simulink model "SNS_GuiCircuit"  (R2025b)
settings: Solver=ode1  StartTime=0.0  StopTime=10.0  FixedStep=0.002  RelTol=1e-3
libraries: SNS_Library x9
Description:
  | SNS network generated from C:\Users\Ben\Documents\GitHub\Bipedal_Robot\Code\Matlab\SNS_Simscape\gui\circuit_last.json. u = input currents nA; S = MN drives in actuator order.
settings Model: Creator=Ben  LastModifiedBy=Ben

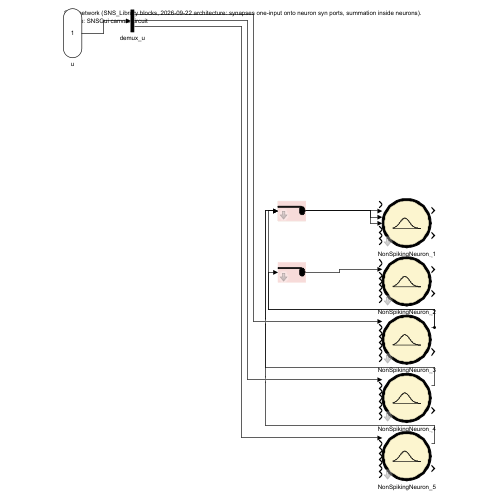
[thumbnail: Simulink's stored preview of the top-level diagram]
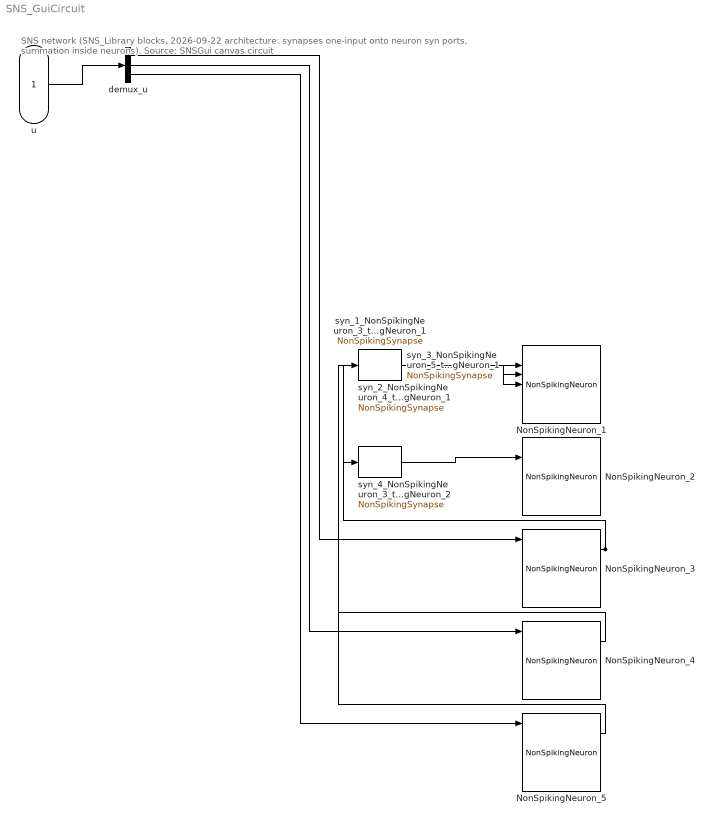
== system SNS_GuiCircuit ==
  note: SNS network (SNS_Library blocks, 2026-09-22 architecture: synapses one-input onto neuron syn ports, summation inside neurons).
      | Source: SNSGui canvas circuit
  u : Inport  PortDimensions=3
  NonSpikingNeuron_{1..5} (5 alike) : SNS_Library/NonSpikingNeuron  Vrest=-52  Gm=0.1  Cm=5  Thr=0  Slope=5
  demux_u : Demux  Outputs=3
  syn_1_NonSpikingNeuron_3_to_NonSpikingNeuron_1 : SNS_Library/NonSpikingSynapse  gmax=1  Esyn=0  ThrPre=-55  SlopePre=1
  syn_2_NonSpikingNeuron_4_to_NonSpikingNeuron_1 : SNS_Library/NonSpikingSynapse  gmax=1  Esyn=-72  ThrPre=-55  SlopePre=1
  syn_3_NonSpikingNeuron_5_to_NonSpikingNeuron_1 : SNS_Library/NonSpikingSynapse  gmax=1  Esyn=-72  ThrPre=-55  SlopePre=1
  syn_4_NonSpikingNeuron_3_to_NonSpikingNeuron_2 : SNS_Library/NonSpikingSynapse  gmax=1  Esyn=-72  ThrPre=-55  SlopePre=1
  wires:
  u/1 -> demux_u/1
  syn_1_NonSpikingNeuron_3_to_NonSpikingNeuron_1/1 -> NonSpikingNeuron_1/2
  syn_2_NonSpikingNeuron_4_to_NonSpikingNeuron_1/1 -> NonSpikingNeuron_1/3
  syn_3_NonSpikingNeuron_5_to_NonSpikingNeuron_1/1 -> NonSpikingNeuron_1/4
  syn_4_NonSpikingNeuron_3_to_NonSpikingNeuron_2/1 -> NonSpikingNeuron_2/2
  demux_u/1 -> NonSpikingNeuron_3/1
  demux_u/2 -> NonSpikingNeuron_4/1
  demux_u/3 -> NonSpikingNeuron_5/1
  NonSpikingNeuron_3/1 -> syn_1_NonSpikingNeuron_3_to_NonSpikingNeuron_1/1, syn_4_NonSpikingNeuron_3_to_NonSpikingNeuron_2/1
  NonSpikingNeuron_4/1 -> syn_2_NonSpikingNeuron_4_to_NonSpikingNeuron_1/1
  NonSpikingNeuron_5/1 -> syn_3_NonSpikingNeuron_5_to_NonSpikingNeuron_1/1
